simulink library "ims_block_library"  (R2018b)
settings: Solver=VariableStepAuto  StartTime=0.0  StopTime=10.0  RelTol=1e-3
undefined symbols (not defined in the file or in its folder): dt_SS_struct, i_t, iA, ss_model, tf_model, Ts
libraries: $bdroot x6
settings Model: Creator=rromano  LastModifiedBy=rromano

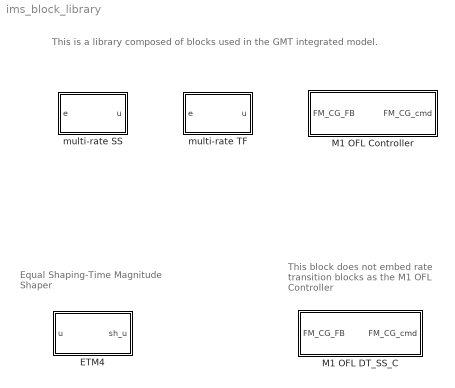
== system ims_block_library ==
  note: This block does not embed rate transition blocks as the M1 OFL Controller
  note: This is a library composed of blocks used in the GMT integrated model.
  note: Equal Shaping-Time Magnitude Shaper
  ETM4 : Subsystem  mask{iA=iA, i_t=i_t, Ts=Ts}
      mask prompts: iA "Impulse Magnitudes"; i_t "Impulse Instants"; Ts "Sampling Time"
      mask DialogControl DescTextVar Prompt: Equal Shaping-Time Magnitude Shaper
  M1 OFL Controller : Subsystem  mask{dt_SS_struct=dt_SS_struct}
      mask prompts: dt_SS_struct "M1 Outer Force Loop Controller (DT SS form)"
  M1 OFL DT_SS_C : Subsystem  mask{dt_SS_struct=dt_SS_struct}
      mask prompts: dt_SS_struct "M1 Outer Force Loop Controller (DT SS form)"
  multi-rate SS : Subsystem  mask{ss_model=ss_model}
      mask prompts: ss_model "Discrete-time state-space model"
      mask DialogControl DescTextVar Prompt: This block is composed of a discrete-time state-space model preceded and followed by a rate-transition to handle the interfaces with different sampling rates.
  multi-rate TF : Subsystem  mask{tf_model=tf_model}
      mask prompts: tf_model "Discrete-time transfer-function model"
      mask DialogControl DescTextVar Prompt: This block is composed of a discrete-time transfer-function model preceded and followed by a rate-transition to handle the interfaces with different sampling rates.

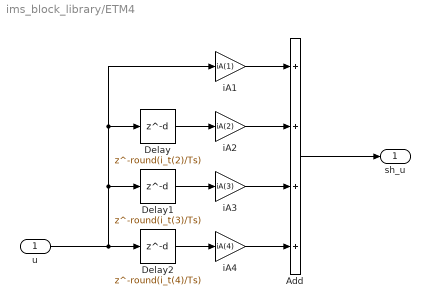
== system ims_block_library/ETM4 ==
  u : Inport
  Add : Sum  Inputs=++++
  Delay : Delay  DelayLength=round(i_t(2)/Ts)  SampleTime=Ts
  Delay1 : Delay  DelayLength=round(i_t(3)/Ts)  SampleTime=Ts
  Delay2 : Delay  DelayLength=round(i_t(4)/Ts)  SampleTime=Ts
  iA1 : Gain  Gain=iA(1)
  iA2 : Gain  Gain=iA(2)
  iA3 : Gain  Gain=iA(3)
  iA4 : Gain  Gain=iA(4)
  sh_u : Outport
  wires:
  iA4/1 -> Add/4
  Delay2/1 -> iA4/1
  iA2/1 -> Add/2
  Delay/1 -> iA2/1
  iA3/1 -> Add/3
  u/1 -> Delay2/1, Delay1/1, iA1/1, Delay/1
  Add/1 -> sh_u/1
  Delay1/1 -> iA3/1
  iA1/1 -> Add/1

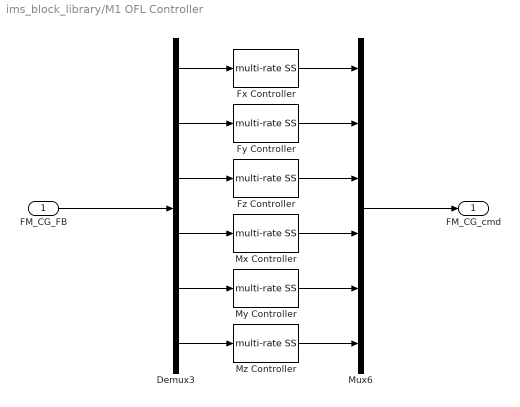
== system ims_block_library/M1 OFL Controller ==
  FM_CG_FB : Inport
  Demux3 : Demux  Outputs=6
  Fx Controller : $bdroot/multi-rate SS  ss_model=dt_SS_struct{1}
  Fy Controller : $bdroot/multi-rate SS  ss_model=dt_SS_struct{2}
  Fz Controller : $bdroot/multi-rate SS  ss_model=dt_SS_struct{3}
  Mux6 : Mux  Inputs=6
  Mx Controller : $bdroot/multi-rate SS  ss_model=dt_SS_struct{4}
  My Controller : $bdroot/multi-rate SS  ss_model=dt_SS_struct{5}
  Mz Controller : $bdroot/multi-rate SS  ss_model=dt_SS_struct{6}
  FM_CG_cmd : Outport
  wires:
  Demux3/6 -> Mz Controller/1
  Demux3/2 -> Fy Controller/1
  Demux3/1 -> Fx Controller/1
  Mux6/1 -> FM_CG_cmd/1
  Demux3/5 -> My Controller/1
  Fz Controller/1 -> Mux6/3
  FM_CG_FB/1 -> Demux3/1
  Demux3/4 -> Mx Controller/1
  Mz Controller/1 -> Mux6/6
  Mx Controller/1 -> Mux6/4
  Fx Controller/1 -> Mux6/1
  Demux3/3 -> Fz Controller/1
  My Controller/1 -> Mux6/5
  Fy Controller/1 -> Mux6/2

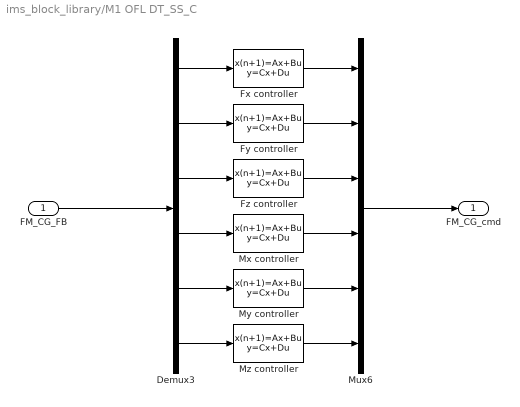
== system ims_block_library/M1 OFL DT_SS_C ==
  FM_CG_FB : Inport
  Demux3 : Demux  Outputs=6
  Fx controller : DiscreteStateSpace  A=dt_SS_struct{1}.A  B=dt_SS_struct{1}.B  C=dt_SS_struct{1}.C  D=dt_SS_struct{1}.D  SampleTime=dt_SS_struct{1}.Ts
  Fy controller : DiscreteStateSpace  A=dt_SS_struct{2}.A  B=dt_SS_struct{2}.B  C=dt_SS_struct{2}.C  D=dt_SS_struct{2}.D  SampleTime=dt_SS_struct{2}.Ts
  Fz controller : DiscreteStateSpace  A=dt_SS_struct{3}.A  B=dt_SS_struct{3}.B  C=dt_SS_struct{3}.C  D=dt_SS_struct{3}.D  SampleTime=dt_SS_struct{3}.Ts
  Mux6 : Mux  Inputs=6
  Mx controller : DiscreteStateSpace  A=dt_SS_struct{4}.A  B=dt_SS_struct{4}.B  C=dt_SS_struct{4}.C  D=dt_SS_struct{4}.D  SampleTime=dt_SS_struct{4}.Ts
  My controller : DiscreteStateSpace  A=dt_SS_struct{5}.A  B=dt_SS_struct{5}.B  C=dt_SS_struct{5}.C  D=dt_SS_struct{5}.D  SampleTime=dt_SS_struct{5}.Ts
  Mz controller : DiscreteStateSpace  A=dt_SS_struct{6}.A  B=dt_SS_struct{6}.B  C=dt_SS_struct{6}.C  D=dt_SS_struct{6}.D  SampleTime=dt_SS_struct{6}.Ts
  FM_CG_cmd : Outport
  wires:
  Mux6/1 -> FM_CG_cmd/1
  FM_CG_FB/1 -> Demux3/1
  Demux3/1 -> Fx controller/1
  Demux3/2 -> Fy controller/1
  Demux3/3 -> Fz controller/1
  Demux3/4 -> Mx controller/1
  Demux3/5 -> My controller/1
  Demux3/6 -> Mz controller/1
  Fx controller/1 -> Mux6/1
  Fy controller/1 -> Mux6/2
  Fz controller/1 -> Mux6/3
  Mx controller/1 -> Mux6/4
  My controller/1 -> Mux6/5
  Mz controller/1 -> Mux6/6

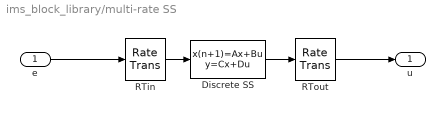
== system ims_block_library/multi-rate SS ==
  e : Inport
  Discrete SS : DiscreteStateSpace  A=ss_model.A  B=ss_model.B  C=ss_model.C  D=ss_model.D  SampleTime=ss_model.Ts
  RTin : RateTransition  OutPortSampleTime=ss_model.Ts
  RTout : RateTransition  OutPortSampleTimeOpt=Inherit
  u : Outport
  wires:
  Discrete SS/1 -> RTout/1
  RTin/1 -> Discrete SS/1
  e/1 -> RTin/1
  RTout/1 -> u/1

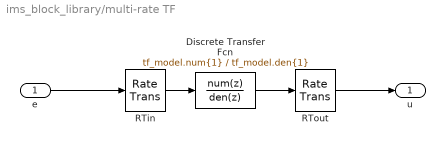
== system ims_block_library/multi-rate TF ==
  e : Inport
  Discrete Transfer Fcn : DiscreteTransferFcn  Numerator=tf_model.num{1}  Denominator=tf_model.den{1}  SampleTime=tf_model.Ts
  RTin : RateTransition  OutPortSampleTime=tf_model.Ts
  RTout : RateTransition  OutPortSampleTimeOpt=Inherit
  u : Outport
  wires:
  e/1 -> RTin/1
  RTout/1 -> u/1
  RTin/1 -> Discrete Transfer Fcn/1
  Discrete Transfer Fcn/1 -> RTout/1
